simulink model "elp_thermal"  (R2026b)
settings: Solver=VariableStepAuto
undefined symbols (not defined in the file or in its folder): P, Ts
libraries: fl_lib x8, nesl_utility x5
settings Model: Creator=aomar  LastModifiedBy=aomar

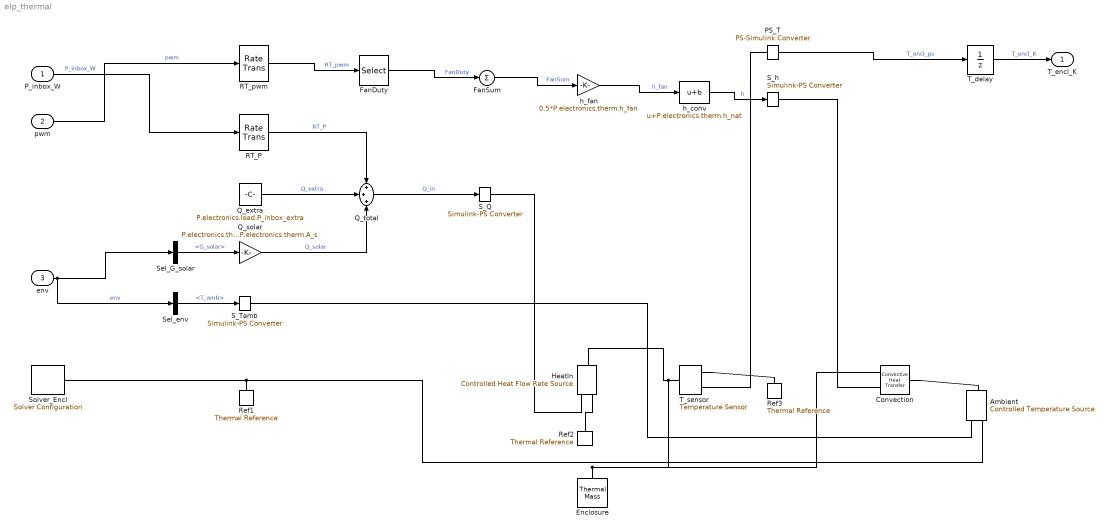
== system elp_thermal ==
  P_inbox_W : Inport  OutDataTypeStr=double  SampleTime=Ts.ctrl
  pwm : Inport  Port=2  OutDataTypeStr=double  PortDimensions=4  SampleTime=Ts.ctrl
  env : Inport  Port=3  OutDataTypeStr=Bus: Bus_EnvState  SampleTime=Ts.hk
  Ambient : fl_lib/Thermal/Thermal Sources/Controlled Temperature Source
  Convection : fl_lib/Thermal/Thermal Elements/Convective Heat Transfer  thermal_type=foundation.enum.constant_variable.variable  area=P.electronics.therm.area m^2  heat_tr_coeff=20 W/(K*m^2)  min_heat_tr_coeff=1e-3 W/(K*m^2)  T_specify=off  T_priority=None  T=0 K  T_nominal_specify=off  T_nominal_value=1  T_nominal_unit=K  Q_specify=off  Q_priority=None  Q=0 W  Q_nominal_specify=off  Q_nominal_value=1  Q_nominal_unit=W
  Enclosure : fl_lib/Thermal/Thermal Elements/Thermal Mass  mass_type=foundation.enum.constant_variable.constant  mass=P.electronics.therm.mass kg  sp_heat=P.electronics.therm.cp J/(kg*K)  mass_min=1e-6 kg  num_ports=foundation.enum.numPorts2.one  m_specify=off  m_priority=High  m=1 kg  m_nominal_specify=off  m_nominal_value=1  m_nominal_unit=kg  T_specify=on  T_priority=High  T=P.electronics.therm.T0 K  T_nominal_specify=off  T_nominal_value=1  T_nominal_unit=K  Q_specify=off  Q_priority=None  Q=0 W  Q_nominal_specify=off  Q_nominal_value=1  Q_nominal_unit=W
  FanDuty : Selector  InputPortWidth=4  IndexOptions=Index vector (dialog)  Indices=[3 4]  OutputSizes=1
  FanSum : Sum  Inputs=+
  HeatIn : fl_lib/Thermal/Thermal Sources/Controlled Heat Flow Rate Source
  PS_T : nesl_utility/PS-Simulink Converter  PhysicalDomain=network_engine_domain  SubClassName=ps_output  LeftPortType=input  RightPortType=output  PseudoPeriodic=off  Frequencies=[]  VectorFormat=inherit  Unit=K  AffineConversion=off
  Q_extra : Constant  Value=P.electronics.load.P_inbox_extra  OutDataTypeStr=double  SampleTime=Ts.hk
  Q_solar : Gain  Gain=P.electronics.therm.alpha_s*P.electronics.therm.A_s
  Q_total : Sum  Inputs=+++
  RT_P : RateTransition  OutPortSampleTime=Ts.hk
  RT_pwm : RateTransition  OutPortSampleTime=Ts.hk
  Ref1 : fl_lib/Thermal/Thermal Elements/Thermal Reference
  Ref2 : fl_lib/Thermal/Thermal Elements/Thermal Reference
  Ref3 : fl_lib/Thermal/Thermal Elements/Thermal Reference
  S_Q : nesl_utility/Simulink-PS Converter  PhysicalDomain=network_engine_domain  SubClassName=ps_input  LeftPortType=input  RightPortType=output  PseudoPeriodic=off  Frequencies=[]  NoiseDistribution=none  NoiseParameters=[]  Unit=W  AffineConversion=off  FilteringAndDerivatives=zero  SimscapeFilterOrder=1  InputFilterTimeConstant=0.001  UdotUserProvided=0
  S_Tamb : nesl_utility/Simulink-PS Converter  PhysicalDomain=network_engine_domain  SubClassName=ps_input  LeftPortType=input  RightPortType=output  PseudoPeriodic=off  Frequencies=[]  NoiseDistribution=none  NoiseParameters=[]  Unit=K  AffineConversion=off  FilteringAndDerivatives=zero  SimscapeFilterOrder=1  InputFilterTimeConstant=0.001  UdotUserProvided=0
  S_h : nesl_utility/Simulink-PS Converter  PhysicalDomain=network_engine_domain  SubClassName=ps_input  LeftPortType=input  RightPortType=output  PseudoPeriodic=off  Frequencies=[]  NoiseDistribution=none  NoiseParameters=[]  Unit=W/(m^2*K)  AffineConversion=off  FilteringAndDerivatives=zero  SimscapeFilterOrder=1  InputFilterTimeConstant=0.001  UdotUserProvided=0
  Sel_G_solar : BusSelector  OutputSignals=G_solar
  Sel_env : BusSelector  OutputSignals=T_amb
  Solver_Encl : nesl_utility/Solver Configuration  PhysicalDomain=network_engine_domain  SubClassName=solver  LeftPortType=input  RightPortType=generic  Tones=[]  Harmonics=[]  SimulateNoise=off  Profile=off  UseLocalSampling=off  EnableSwitchedLinearOptims=on  FrequencyDomain=off  UseCCode=off  RelTol=0.001  AbsTol=0.001  MinStep=1e-09  ToWorkspace=off  RevertToSquareIcSolve=off  NumHomotopyIterations=100  PhasorMode=off  PhasorModeNumHarmonics=1  ConsistencySolver=NEWTON_XTOL_AFTER_FTOL  CanonicalOrdering=CANONICAL  OptimizeIntermediates=OPTIMIZED  MulticoreSolverChoice=BACKWARD_EULER  IndexReductionMethod=DerivativeReplacement  DoDC=off  ResidualTolerance=1e-09  ConsistencyTolSource=GLOBAL  ConsistencyAbsTol=0.001  ConsistencyRelTol=0.001  ConsistencyTolFactor=0.001  UseLocalSolver=on  LocalSolverChoice=NE_BACKWARD_EULER_ADVANCER  ResolveIndetEquations=on  FunctionEvalNumThread=1  LocalSolverSampleTime=P.sim.ssc.Ts_encl  DoFixedCost=on  MaxNonlinIter=3  MaxModeIter=2  ComputeImpulses=off  ImpulseIterations=2  LinearAlgebra=auto  LinearAlgebraNumThread=0  EquationFormulation=NE_TIME_EF  DelaysMemoryBudget=1024  AutomaticFiltering=on  FilteringTimeConstant=0.001  PartitionStorageMethod=AS_NEEDED  PartitionMemoryBudget=1024  PartitionMethod=BALANCED  MultibodyUseLocalSolver=off  MultibodyLocalSolverChoice=ODE1  MultibodyLocalSolverSampleTime=0.001
  T_delay : UnitDelay  InitialCondition=P.electronics.therm.T0  SampleTime=Ts.hk
  T_sensor : fl_lib/Thermal/Thermal Sensors/Temperature Sensor  temperature_measure=foundation.enum.MeasurementReference.difference
  h_conv : Bias  Bias=P.electronics.therm.h_nat  SaturateOnIntegerOverflow=off
  h_fan : Gain  Gain=0.5*P.electronics.therm.h_fan
  T_encl_K : Outport  OutDataTypeStr=double
  wires:
  P_inbox_W/1 -> RT_P/1  "P_inbox_W"
  pwm/1 -> RT_pwm/1  "pwm"
  env/1 -> Sel_G_solar/1, Sel_env/1  "env"
  Sel_G_solar/1 -> Q_solar/1  "<G_solar>"
  Sel_env/1 -> S_Tamb/1  "<T_amb>"
  Q_extra/1 -> Q_total/2  "Q_extra"
  Q_solar/1 -> Q_total/3  "Q_solar"
  RT_pwm/1 -> FanDuty/1  "RT_pwm"
  RT_P/1 -> Q_total/1  "RT_P"
  Q_total/1 -> S_Q/1  "Q_in"
  FanDuty/1 -> FanSum/1  "FanDuty"
  FanSum/1 -> h_fan/1  "FanSum"
  h_fan/1 -> h_conv/1  "h_fan"
  h_conv/1 -> S_h/1  "h"
  PS_T/1 -> T_delay/1  "T_encl_ps"
  T_delay/1 -> T_encl_K/1  "T_encl_K"
  connections:
  Convection/RConn1 -- Ambient/LConn1
  S_Tamb/RConn1 -- Ambient/RConn1
  Ref1/LConn1 -- Solver_Encl/RConn1 -- Ambient/RConn2
  S_h/RConn1 -- Convection/LConn2
  S_Q/RConn1 -- HeatIn/RConn1
  HeatIn/RConn2 -- Ref2/LConn1
  PS_T/LConn1 -- T_sensor/RConn2
  T_sensor/LConn1 -- HeatIn/LConn1 -- Enclosure/LConn1 -- Convection/LConn1
  T_sensor/RConn1 -- Ref3/LConn1
